simulink model "DKE"  (R2026b)
settings: Solver=ode4  StopTime=1000  FixedStep=1e-2
values from neighbouring files (symbols this model uses):
  a = R_e + h    (= 8000000)    [DKE_Parameters.m]    (also in disturbances_validation.m)
  A0 = eye(3)    [DKE_Parameters.m]    (also in disturbances_validation.m)
  A_body1_4 = 0.082716    [DKE_Parameters.m]    (also in disturbances_validation.m)
  A_body5_6 = 0.051076    [DKE_Parameters.m]    (also in disturbances_validation.m)
  A_panel = 0.0544    [DKE_Parameters.m]    (also in disturbances_validation.m)
  B1 = [+1; 0; 0]    [DKE_Parameters.m]    (also in disturbances_validation.m)
  B2 = [-1; 0; 0]    [DKE_Parameters.m]    (also in disturbances_validation.m)
  Bias_static = [1.8; -1.8; 1.8] * (1/3600) * (pi/180)    [DKE_Parameters.m]
  cos_FoV = cosd(FoV_half_deg)    [DKE_Parameters.m]
  e = 0.01    [DKE_Parameters.m]    (also in disturbances_validation.m = 0)
  epsilon = deg2rad(23.45)    [DKE_Parameters.m]    (also in disturbances_validation.m)
  f = 0.05    [DKE_Parameters.m]
  G = 6.67E-11    (= 6.67e-11)    [DKE_Parameters.m]    (also in disturbances_validation.m)
  H0 = sqrt(g10^2 + g11^2 + h11^2)    [DKE_Parameters.m]    (also in disturbances_validation.m)
  i = deg2rad(45)    [DKE_Parameters.m]    (also in disturbances_validation.m = deg2rad(0))
  I_depl = [Ixx, Ixy, Ixz ... (first row only)    [DKE_Parameters.m]    (also in disturbances_validation.m = diag([  Ix,   Iy,   Iz]))
  I_inv = I_depl \ eye(size(I_depl))    [DKE_Parameters.m]    (also in disturbances_validation.m = diag([1/Ix, 1/Iy, 1/Iz]))
  Ixx = 22.53E-2    (= 0.2253)    [DKE_Parameters.m]
  Iyy = 26.71E-2    (= 0.2671)    [DKE_Parameters.m]
  Izz = 33.03E-2    (= 0.3303)    [DKE_Parameters.m]
  j_B = [0.01; 0.05; 0.01]    [DKE_Parameters.m]    (also in disturbances_validation.m = [0 0 0])
  L1 = [0; 0; +1]    [DKE_Parameters.m]    (also in disturbances_validation.m)
  L2 = [0; +1; 0]    [DKE_Parameters.m]    (also in disturbances_validation.m)
  L3 = [0; 0; -1]    [DKE_Parameters.m]    (also in disturbances_validation.m)
  L4 = [0; -1; 0]    [DKE_Parameters.m]    (also in disturbances_validation.m)
  M_e = 5.97E24    (= 5.97e+24)    [DKE_Parameters.m]    (also in disturbances_validation.m)
  M_misalign = [1,  g_xy,  g_xz ... (first row only)    [DKE_Parameters.m]
  n_e = sqrt(mu_e/a^3)    [DKE_Parameters.m]
  n_s = 2*pi/T_s    (= 1.99102127766e-07)    [DKE_Parameters.m]    (also in disturbances_validation.m)
  omega = [0; 0; 0]    [disturbances_validation.m]
  omega_0 = [0.02; 0.05; 0.08]    [DKE_Parameters.m]
  omega_e = 2*pi/T_e    (= 7.29212351699e-05)    [DKE_Parameters.m]
  P = J_s/c    (= 4.52666666667e-06)    [DKE_Parameters.m]    (also in Panel_inertia_calc.m = 4.56e-06; disturbances_validation.m)
  Panel1 = [+1; 0; 0]    [DKE_Parameters.m]    (also in disturbances_validation.m)
  Panel2 = [+1; 0; 0]    [DKE_Parameters.m]    (also in disturbances_validation.m)
  Panel3 = [-1; 0; 0]    [DKE_Parameters.m]    (also in disturbances_validation.m)
  Panel4 = [-1; 0; 0]    [DKE_Parameters.m]    (also in disturbances_validation.m)
  r_CM = [0.015; 0.02; 0]    [DKE_Parameters.m]    (also in disturbances_validation.m = [0; 0; 0])
  R_e = 6371E3    (= 6371000)    [DKE_Parameters.m]
  r_s = 1.496E11    (= 149600000000)    [DKE_Parameters.m]
  rF1 = [0; 0; +0.113]    [DKE_Parameters.m]    (also in disturbances_validation.m)
  rF10 = [0; -0.273; 0]    [DKE_Parameters.m]    (also in disturbances_validation.m)
  rF2 = [0; +0.113; 0]    [DKE_Parameters.m]    (also in disturbances_validation.m)
  rF3 = [0; 0; -0.113]    [DKE_Parameters.m]    (also in disturbances_validation.m)
  rF4 = [0; -0.113; 0]    [DKE_Parameters.m]    (also in disturbances_validation.m)
  rF5 = [+0.183; 0; 0]    [DKE_Parameters.m]    (also in disturbances_validation.m)
  rF6 = [-0.183; 0; 0]    [DKE_Parameters.m]    (also in disturbances_validation.m)
  rF7 = [0; +0.273; 0]    [DKE_Parameters.m]    (also in disturbances_validation.m)
  rF8 = [0; -0.273; 0]    [DKE_Parameters.m]    (also in disturbances_validation.m)
  rF9 = [0; +0.273; 0]    [DKE_Parameters.m]    (also in disturbances_validation.m)
  rho_d = 0.1    [DKE_Parameters.m]    (also in disturbances_validation.m)
  rho_s_body = 0.5    [DKE_Parameters.m]    (also in disturbances_validation.m)
  rho_s_panel = 0.1    [DKE_Parameters.m]    (also in disturbances_validation.m)
  S_catalog = S_all    [DKE_Parameters.m]
  S_T = S_catalog'    [DKE_Parameters.m]
  S_tilde = A_e * S_catalog    [DKE_Parameters.m]
  Scale_factor = [500; -450; 300]    [DKE_Parameters.m]
  seed_u = randi(1000000, 1, N_stars)    [DKE_Parameters.m]
  seed_v = randi(1000000, 1, N_stars) + 1    [DKE_Parameters.m]
  theta_0 = deg2rad(100)    [DKE_Parameters.m]
  tilt_mag = deg2rad(11.5)    [DKE_Parameters.m]    (also in disturbances_validation.m = deg2rad(0))
  Ts = 0.01    [DKE_Parameters.m]
  var_uv = (f * tan(sigma_rad))^2    [DKE_Parameters.m]
undefined symbols (not defined in the file or in its folder): DiscIntNeverNeededParam
libraries: matrix_library x13, simulink x3
(part 2 of 2)

== system DKE/Environment/Orbital propagation/theta_dot/Theta_dot ==
  Ecc : Inport
  cos(theta) : Inport  Port=2
  Constant : Constant  Value=n_e
  Constant1 : Constant  Value=theta_0
  Constant2 : Constant
  Constant5 : Constant  Value=3/2
  Divide1 : Product  Inputs=*/
  Integrator : Integrator  InitialConditionSource=external
  Math Function : Math  Operator=square
  Math Function1 : Math  Operator=square
  Power : Math  Operator=pow
  Product5 : Product
  Product6 : Product
  Subtract : Sum  Inputs=+-
  Sum2 : Sum  Inputs=|++
  Theta : Outport
  wires:
  Ecc/1 -> Math Function/1, Product6/1
  Product6/1 -> Sum2/2
  Constant1/1 -> Integrator/2
  Subtract/1 -> Power/1
  Math Function1/1 -> Product5/2
  Constant2/1 -> Sum2/1, Subtract/1
  Power/1 -> Divide1/2
  Product5/1 -> Divide1/1
  Constant5/1 -> Power/2
  Sum2/1 -> Math Function1/1
  Constant/1 -> Product5/1
  Divide1/1 -> Integrator/1  "theta_dot"
  Integrator/1 -> Theta/1  "theta"
  cos(theta)/1 -> Product6/2
  Math Function/1 -> Subtract/2

== system DKE/Environment/Orbital propagation/theta_dot/r_hat ==
  theta : Inport
  Cos1 : Trigonometry  Operator=cos
  Cos2 : Trigonometry  Operator=cos
  Mux : Mux  Inputs=3
  Product3 : Product
  Product4 : Product
  Sin : Trigonometry
  Sin1 : Trigonometry
  inclination : Constant  Value=i
  r_hat : Outport
  wires:
  Product4/1 -> Mux/2  "Y"
  Product3/1 -> Mux/3  "Z"
  Cos1/1 -> Product4/2
  Sin1/1 -> Product3/2
  inclination/1 -> Sin1/1, Cos1/1
  Mux/1 -> r_hat/1  "3x1"
  Cos2/1 -> Mux/1  "X"
  Sin/1 -> Product4/1, Product3/1
  theta/1 -> Cos2/1, Sin/1
